simulink model "MAIN"  (R2023a)
settings: Solver=ode45  StartTime=0.0  StopTime=100  RelTol=1e-3
libraries: slpidlib x2
settings Model: Creator=james  LastModifiedBy=james

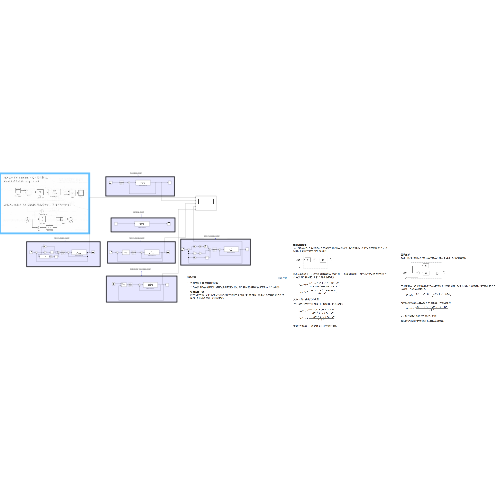
[thumbnail: Simulink's stored preview of the top-level diagram]
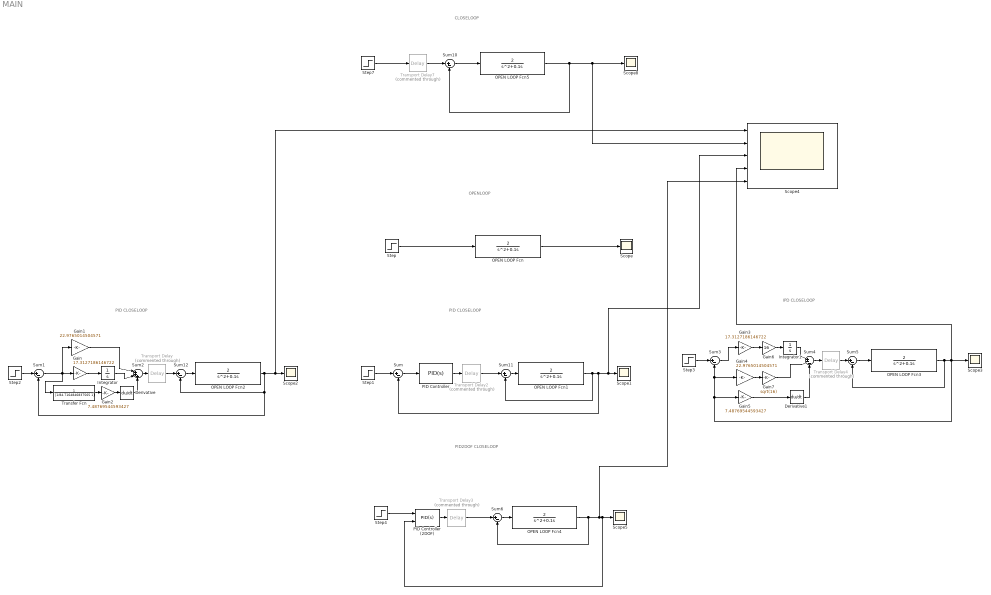
== system MAIN ==
  note: OPENLOOP
  note: PID CLOSELOOP
  note: PID CLOSELOOP
  note: IPD CLOSELOOP
  note: PID2DOF CLOSELOOP
  note: CLOSELOOP
  Derivative : Derivative
  Derivative1 : Derivative
  Gain : Gain  Gain=17.3127186146722
  Gain1 : Gain  Gain=22.9765014504571
  Gain2 : Gain  Gain=7.48769544593427
  Gain3 : Gain  Gain=17.3127186146722
  Gain4 : Gain  Gain=22.9765014504571
  Gain5 : Gain  Gain=7.48769544593427
  Gain6 : Gain  Gain=16
  Gain7 : Gain  Gain=sqrt(16)
  Integrator : Integrator
  Integrator1 : Integrator
  OPEN LOOP Fcn{,1..5} (6 alike) : TransferFcn  Numerator=[2]  Denominator=[1 0.1 0]
  PID Controller : slpidlib/PID Controller  Controller=PID  Form=Parallel  TimeDomain=Continuous-time  UseExternalTs=off  SampleTime=-1  IntegratorMethod=Forward Euler  FilterMethod=Forward Euler  ControllerParametersSource=internal  P=22.9765014504571  I=17.3127186146722  UseKiTs=on  D=7.48769544593427  N=84.7164846837565  UseFilter=on  TunerSelectOption=Transfer Function Based (PID Tuner App)  InitialConditionSource=internal  InitialConditionForIntegrator=0  InitialConditionForFilter=0  DifferentiatorICPrevScaledInput=0  ExternalReset=none  TrackingMode=off  Kt=1  LimitOutput=off  SatLimitsSource=internal  UpperSaturationLimit=inf  LowerSaturationLimit=-inf  LinearizeAsGain=on  AntiWindupMode=none  Kb=1  LimitIntegrator=off  UpperIntegratorSaturationLimit=inf  LowerIntegratorSaturationLimit=-inf  POutMin=[]  POutMax=[]  IOutMin=[]  IOutMax=[]  DOutMin=[]  DOutMax=[]  NOutMin=[]  NOutMax=[]  SumOutMin=[]  SumOutMax=[]  SaturationOutMin=[]  SaturationOutMax=[]  PParamMin=[]  PParamMax=[]  IParamMin=[]  IParamMax=[]  DParamMin=[]  DParamMax=[]  NParamMin=[]  NParamMax=[]  KbParamMin=[]  KbParamMax=[]  KtParamMin=[]  KtParamMax=[]  KbOutMin=[]  KbOutMax=[]  KtOutMin=[]  KtOutMax=[]  IntegratorOutMin=[]  IntegratorOutMax=[]  FilterOutMin=[]  FilterOutMax=[]  SumI1OutMin=[]  SumI1OutMax=[]  SumI2OutMin=[]  SumI2OutMax=[]  SumI3OutMin=[]  SumI3OutMax=[]  SumI4OutMin=[]  SumI4OutMax=[]  SumDOutMin=[]  SumDOutMax=[]  DifferentiatorOutMin=[]  DifferentiatorOutMax=[]  FilterDiffOutCoefMin=[]  FilterDiffOutCoefMax=[]  ReciprocalOutMin=[]  ReciprocalOutMax=[]  SumDenOutMin=[]  SumDenOutMax=[]  SumNumOutMin=[]  SumNumOutMax=[]  DivideOutMin=[]  DivideOutMax=[]  UdiffTsProdOutMin=[]  UdiffTsProdOutMax=[]  NTsProdOutMin=[]  NTsProdOutMax=[]  UintegralTsProdOutMin=[]  UintegralTsProdOutMax=[]  UngainTsProdOutMin=[]  UngainTsProdOutMax=[]  ClampingZeroOutDataTypeStr=Inherit: Inherit via back propagation  ClampingZeroOutMin=[]  ClampingZeroOutMax=[]  FilterDenConstantOutDataTypeStr=Inherit: Inherit via back propagation  FilterDenConstantOutMin=[]  FilterDenConstantOutMax=[]  PCopyOutDataTypeStr=Inherit: Inherit via back propagation  PCopyOutMin=[]  PCopyOutMax=[]  NCopyOutDataTypeStr=Inherit: Inherit via back propagation  NCopyOutMin=[]  NCopyOutMax=[]  IntegratorContinuousStateAttributes=''  IntegratorStateMustResolveToSignalObject=off  IntegratorRTWStateStorageClass=Auto  FilterContinuousStateAttributes=''  FilterStateMustResolveToSignalObject=off  FilterRTWStateStorageClass=Auto  ParallelPVariant=InternalParameters  IdealPVariant=Disabled  IVariant=InternalParameters  DVariant=InternalParameters  IntegratorVariant=Continuous  SatVariant=Disabled  AWVariant=Passthrough  PCopyVariant=Disabled  TRVariant=Disabled  FdbkBlocksVariant=Forward  IdealPFdbkVariant=Disabled  SatFdbkVariant=Disabled  DerivativeFilterVariant=ContFilter  NVariant=InternalParameters  NCopyVariant=Disabled  FilterICVariant=InternalICsFilter  IntegratorICVariant=InternalICs  ExternalResetVariant=Disabled  TRSumVariant=Passthrough  SumFdbkVariant=Disabled  SumVariant=Sum_PID  TsampFilterVariant=InternalTs  TsampNgainVariant=Passthrough  TsampIntegralVariant=Disabled_SignalSpec  ExternalSaturationOutDataTypeStr=Inherit: Same as second input
  PID Controller (2DOF) : slpidlib/PID Controller (2DOF)  Controller=PID  Form=Parallel  TimeDomain=Continuous-time  UseExternalTs=off  SampleTime=-1  IntegratorMethod=Forward Euler  FilterMethod=Forward Euler  ControllerParametersSource=internal  P=15.9453197302959  I=10.062511985101  UseKiTs=on  D=6.20248231367413  N=70.464102775123  UseFilter=on  b=0.985272444154741  c=0.717949850740547  TunerSelectOption=Transfer Function Based (PID Tuner App)  InitialConditionSource=internal  InitialConditionForIntegrator=0  InitialConditionForFilter=0  DifferentiatorICPrevScaledInput=0  ExternalReset=none  TrackingMode=off  Kt=1  LimitOutput=off  SatLimitsSource=internal  UpperSaturationLimit=inf  LowerSaturationLimit=-inf  LinearizeAsGain=on  AntiWindupMode=none  Kb=1  LimitIntegrator=off  UpperIntegratorSaturationLimit=inf  LowerIntegratorSaturationLimit=-inf  POutMin=[]  POutMax=[]  IOutMin=[]  IOutMax=[]  DOutMin=[]  DOutMax=[]  NOutMin=[]  NOutMax=[]  bOutMin=[]  bOutMax=[]  cOutMin=[]  cOutMax=[]  SumOutMin=[]  SumOutMax=[]  SaturationOutMin=[]  SaturationOutMax=[]  PParamMin=[]  PParamMax=[]  IParamMin=[]  IParamMax=[]  DParamMin=[]  DParamMax=[]  NParamMin=[]  NParamMax=[]  bParamMin=[]  bParamMax=[]  cParamMin=[]  cParamMax=[]  KbParamMin=[]  KbParamMax=[]  KtParamMin=[]  KtParamMax=[]  KbOutMin=[]  KbOutMax=[]  KtOutMin=[]  KtOutMax=[]  IntegratorOutMin=[]  IntegratorOutMax=[]  FilterOutMin=[]  FilterOutMax=[]  SumI1OutMin=[]  SumI1OutMax=[]  SumI2OutMin=[]  SumI2OutMax=[]  SumI3OutMin=[]  SumI3OutMax=[]  SumI4OutMin=[]  SumI4OutMax=[]  SumDOutMin=[]  SumDOutMax=[]  Sum1OutMin=[]  Sum1OutMax=[]  Sum2OutMin=[]  Sum2OutMax=[]  Sum3OutMin=[]  Sum3OutMax=[]  DifferentiatorOutMin=[]  DifferentiatorOutMax=[]  FilterDiffOutCoefMin=[]  FilterDiffOutCoefMax=[]  ReciprocalOutMin=[]  ReciprocalOutMax=[]  SumDenOutMin=[]  SumDenOutMax=[]  SumNumOutMin=[]  SumNumOutMax=[]  DivideOutMin=[]  DivideOutMax=[]  UdiffTsProdOutMin=[]  UdiffTsProdOutMax=[]  NTsProdOutMin=[]  NTsProdOutMax=[]  UintegralTsProdOutMin=[]  UintegralTsProdOutMax=[]  UngainTsProdOutMin=[]  UngainTsProdOutMax=[]  ClampingZeroOutDataTypeStr=Inherit: Inherit via back propagation  ClampingZeroOutMin=[]  ClampingZeroOutMax=[]  FilterDenConstantOutDataTypeStr=Inherit: Inherit via back propagation  FilterDenConstantOutMin=[]  FilterDenConstantOutMax=[]  PCopyOutDataTypeStr=Inherit: Inherit via back propagation  PCopyOutMin=[]  PCopyOutMax=[]  NCopyOutDataTypeStr=Inherit: Inherit via back propagation  NCopyOutMin=[]  NCopyOutMax=[]  IntegratorContinuousStateAttributes=''  IntegratorStateMustResolveToSignalObject=off  IntegratorRTWStateStorageClass=Auto  FilterContinuousStateAttributes=''  FilterStateMustResolveToSignalObject=off  FilterRTWStateStorageClass=Auto  ParallelPVariant=InternalParameters  IdealPVariant=Disabled  IVariant=InternalParameters  DVariant=InternalParameters  bVariant=InternalParameters  cVariant=InternalParameters  IntegratorVariant=Continuous  SatVariant=Disabled  AWVariant=Passthrough  PCopyVariant=Disabled  TRVariant=Disabled  FdbkBlocksVariant=Forward  IdealPFdbkVariant=Disabled  SatFdbkVariant=Disabled  DerivativeFilterVariant=ContFilter  NVariant=InternalParameters  NCopyVariant=Disabled  FilterICVariant=InternalICsFilter  IntegratorICVariant=InternalICs  ExternalResetVariant=Disabled  TRSumVariant=Passthrough  SumFdbkVariant=Disabled  SumVariant=Sum_PID  TsampFilterVariant=InternalTs  TsampNgainVariant=Passthrough  TsampIntegralVariant=Disabled_SignalSpec  ExternalSaturationOutDataTypeStr=Inherit: Same as second input
  Scope{,1..3,5,8} (6 alike) : Scope
  Scope4 : Scope  NumInputPorts=5
  Step{,1..4,7} (6 alike) : Step  SampleTime=0
  Sum{,1,3,5..6,10..12} (8 alike) : Sum  Inputs=|+-
  Sum2 : Sum  Inputs=|+++
  Sum4 : Sum  Inputs=|+--
  Transfer Fcn : TransferFcn  Denominator=[1/84.7164846837565 1]
  Transport Delay{,2..4,7} (5 alike) : TransportDelay  Commented=through  DelayTime=0.1
  wires:
  Step/1 -> OPEN LOOP Fcn/1
  PID Controller/1 -> Transport Delay2/1
  OPEN LOOP Fcn1/1 -> Sum11/2, Sum/2, Scope4/3, Scope1/1
  Step1/1 -> Sum/1
  Sum/1 -> PID Controller/1
  Sum1/1 -> Transfer Fcn/1, Gain1/1, Gain/1
  Integrator/1 -> Sum2/2
  Step2/1 -> Sum1/1
  Gain/1 -> Integrator/1
  Gain2/1 -> Derivative/1
  Derivative/1 -> Sum2/3
  Sum2/1 -> Transport Delay/1
  Gain1/1 -> Sum2/1
  Gain3/1 -> Gain6/1
  Sum3/1 -> Gain3/1
  Integrator1/1 -> Sum4/1
  OPEN LOOP Fcn3/1 -> Sum5/2, Gain5/1, Gain4/1, Sum3/2, Scope4/4, Scope3/1
  Sum4/1 -> Transport Delay4/1
  Step3/1 -> Sum3/1
  Derivative1/1 -> Sum4/3
  Gain4/1 -> Gain7/1
  OPEN LOOP Fcn2/1 -> Sum12/2, Sum1/2, Scope4/1, Scope2/1
  Gain6/1 -> Integrator1/1
  Gain7/1 -> Sum4/2
  Gain5/1 -> Derivative1/1
  PID Controller (2DOF)/1 -> Transport Delay3/1
  Step4/1 -> PID Controller (2DOF)/1
  OPEN LOOP Fcn4/1 -> Sum6/2, PID Controller (2DOF)/2, Scope5/1, Scope4/5
  Transport Delay/1 -> Sum12/1
  OPEN LOOP Fcn/1 -> Scope/1
  Transport Delay2/1 -> Sum11/1
  Transport Delay3/1 -> Sum6/1
  Transport Delay4/1 -> Sum5/1
  Step7/1 -> Transport Delay7/1
  OPEN LOOP Fcn5/1 -> Sum10/2, Scope4/2, Scope8/1
  Sum10/1 -> OPEN LOOP Fcn5/1
  Transport Delay7/1 -> Sum10/1
  Sum11/1 -> OPEN LOOP Fcn1/1
  Sum12/1 -> OPEN LOOP Fcn2/1
  Sum5/1 -> OPEN LOOP Fcn3/1
  Sum6/1 -> OPEN LOOP Fcn4/1
  Transfer Fcn/1 -> Gain2/1
